simulink model "sm_car_"  (R2026b)
settings: Solver=ode23t  StopTime=100  MaxStep=0.4  AbsTol=1e-3  EnableMultiTasking=on
PreLoadFcn:
  | % Due to usability issue in Repeating Sequence block
  | warning('off','Simulink:Masking:Invalid');
  | 
  | % Eliminate unnecessary warnings in inactive variants
  | % Warnings generated only if you click through inactive variant
  | warning('off','MATLAB:nonExistentField');
  | warning('off','Simulink:Parameters:BlkParamUndefined');
PostLoadFcn:
  | set_param([bdroot '/Vehicle'],'popup_trailer','Off')
  | warning('off','sm:sli:setup:compile:LocalSolverNotSupported')
  | %sm_car_config_maneuver(bdroot,'WOT Braking');
  | sm_car_config_vehicle(bdroot,'false');
  | sm_car_config_logging(bdroot);
InitFcn:
  | sm_car_config_camera;
  | Vehicle = sm_car_vehcfg_checkConfig(Vehicle);
  | sm_car_check_tire_model(bdroot);
StartFcn:
  | tic;
StopFcn:
  | Elapsed_Sim_Time = toc;
  | % disp(['Elapsed Sim Time = ' num2str(Elapsed_Sim_Time)]);
undefined symbols (not defined in the file or in its folder): acc_theta, accel_ramp_rate, Axle1D, AxleIn, Camera, Control, Driver, Init, Maneuver, Pedal, Scene, ShaftL1, ShaftL2, ShaftR1, ShaftR2, Visual, X, xy_data_car_side, Y, Z
libraries: sm_lib x290, fl_lib x171, nesl_utility x144, simulink x60, simulink_extras x14, sdl_lib x14, SimscapeFluids_lib x7, Damper_Element x4, Tire_1x2x x4, ee_lib x3, Scene_Utilities x3, sharedTrackingLibrary x2
(part 10 of 22)

== system sm_car_/Driver/Closed Loop1/Override/None ==
  dist : Inport
  Obs : Inport  Port=2
  Bus Creator{,2..4} (4 alike) : BusCreator  Inputs=2
  Bus Creator1 : BusCreator  Inputs=4
  Constant{1..2,4,6} (4 alike) : Constant  Value=0
  Constant{3,5,7..8} (4 alike) : Constant
  Terminator : Terminator
  Terminator1 : Terminator
  Ovr : Outport  VectorParamsAs1DForOutWhenUnconnected=off
  wires:
  dist/1 -> Terminator/1
  Obs/1 -> Terminator1/1
  Bus Creator1/1 -> Ovr/1
  Constant1/1 -> Bus Creator/1  "offset"
  Constant8/1 -> Bus Creator/2  "gain"
  Constant6/1 -> Bus Creator4/1  "offset"
  Constant7/1 -> Bus Creator4/2  "gain"
  Constant5/1 -> Bus Creator3/2  "gain"
  Constant4/1 -> Bus Creator3/1  "offset"
  Constant3/1 -> Bus Creator2/2  "gain"
  Bus Creator2/1 -> Bus Creator1/3  "z"
  Constant2/1 -> Bus Creator2/1  "offset"
  Bus Creator3/1 -> Bus Creator1/2  "y"
  Bus Creator/1 -> Bus Creator1/4  "vx"
  Bus Creator4/1 -> Bus Creator1/1  "x"

== system sm_car_/Vehicle/Vehicle/Body to World/R to X-Y-Z Extrinsic ==
  note: The sensor implemented here computes roll / pitch / yaw values assuming they correpsond to X, Y, and Z rotations, applied in that order and using  *extrinsic* rotations.  That is, the rotations are applied about the fixed (non-rotated) axes of the base frame.   There are many other possible conventions, but the computations of angles has the same basic structure for any of them.  The only differences would be which elements of the rotation matrix are picked off for analysis, and which signals are negated.
      |
      | This implementation does not handle the gimbal-lock case robustly, which occurs when the Y (pitch) rotation is +/-90 degrees.  Handling this case requires a more complex computation,
      | but it can be done with a few more trig blocks and selectors.
  R : Inport
  Asin : Trigonometry  Operator=asin
  Atan1 : Trigonometry  Operator=atan2
  Atan2 : Trigonometry  Operator=atan2
  Demux : Demux  Outputs=2
  Demux1 : Demux  Outputs=2
  Multiply2 : Gain  Gain=-1
  "R(3, 1)" : Selector  NumberOfDimensions=2  InputPortWidth=3  IndexOptions=Index vector (dialog),Index vector (dialog)  Indices=3,1  OutputSizes=1,1  RuntimeRangeChecks=off
  "R(3, 2:3)" : Selector  NumberOfDimensions=2  InputPortWidth=3  IndexOptions=Index vector (dialog),Index vector (dialog)  Indices=3,[2 3]  OutputSizes=1,1  RuntimeRangeChecks=off
  "R([2 1], 1)" : Selector  NumberOfDimensions=2  InputPortWidth=3  IndexOptions=Index vector (dialog),Index vector (dialog)  Indices=[2 1],1  OutputSizes=1,1  RuntimeRangeChecks=off
  Reshape : Reshape
  Reshape1 : Reshape
  Reshape2 : Reshape  OutputDimensionality=Customize  OutputDimensions=1
  yaw : Outport  VectorParamsAs1DForOutWhenUnconnected=off
  pitch : Outport  Port=2  VectorParamsAs1DForOutWhenUnconnected=off
  roll : Outport  Port=3  VectorParamsAs1DForOutWhenUnconnected=off
  wires:
  Reshape2/1 -> roll/1
  Reshape1/1 -> pitch/1
  Reshape/1 -> yaw/1
  Atan1/1 -> Reshape/1
  "R(3, 2:3)"/1 -> Demux/1
  Multiply2/1 -> Asin/1
  "R([2 1], 1)"/1 -> Demux1/1
  Demux1/1 -> Atan1/1
  R/1 -> "R([2 1], 1)"/1, "R(3, 2:3)"/1, "R(3, 1)"/1
  Asin/1 -> Reshape1/1
  "R(3, 1)"/1 -> Multiply2/1
  Atan2/1 -> Reshape2/1
  Demux/2 -> Atan2/2
  Demux1/2 -> Atan1/2
  Demux/1 -> Atan2/1

== system sm_car_/Vehicle/Vehicle/Brakes/PedalAbstract DiscDisc ==
  In Bus Element5 : Inport  PortName=DrvBus  Element=rBrakePedal
  In Bus Element1 : Inport  Port=2  PortName=CtrlBus
  Actuator L1 : Subsystem  mask(Brake Actuator, Pedal Input){brk_max_p=brk_max_p_a1, brk_filt=brk_filt_a1}
      mask prompts: brk_max_p "Max Pad Pressure (Pa)"; brk_filt "Time Constant (s)"
      mask help: Models brake actuator dynamics. A transfer function models delay from brake pedal movement to pressure applied at brake rotor.
      mask TypeOptions brk_max_p: Filter/Numerator
  Actuator L2 : Subsystem  mask(Brake Actuator, Pedal Input){brk_max_p=brk_max_p_a2, brk_filt=brk_filt_a2}
      mask prompts: brk_max_p "Max Pad Pressure (Pa)"; brk_filt "Time Constant (s)"
      mask help: Models brake actuator dynamics. A transfer function models delay from brake pedal movement to pressure applied at brake rotor.
      mask TypeOptions brk_max_p: Filter/Numerator
  Actuator R1 : Subsystem  mask(Brake Actuator, Pedal Input){brk_max_p=brk_max_p_a1, brk_filt=brk_filt_a1}
      mask prompts: brk_max_p "Max Pad Pressure (Pa)"; brk_filt "Time Constant (s)"
      mask help: Models brake actuator dynamics. A transfer function models delay from brake pedal movement to pressure applied at brake rotor.
      mask TypeOptions brk_max_p: Filter/Numerator
  Actuator R2 : Subsystem  mask(Brake Actuator, Pedal Input){brk_max_p=brk_max_p_a2, brk_filt=brk_filt_a2}
      mask prompts: brk_max_p "Max Pad Pressure (Pa)"; brk_filt "Time Constant (s)"
      mask help: Models brake actuator dynamics. A transfer function models delay from brake pedal movement to pressure applied at brake rotor.
      mask TypeOptions brk_max_p: Filter/Numerator
  Disc Brake L1 : sdl_lib/Brakes & Detents/Rotational/Disc Brake  r_mean=brk_pad_rad_a1 m  bore=brk_cyl_bore_a1 m  n_pads=brk_n_pads_a1  thermal_port=simscape.enum.thermaleffects.omit  mu_static=brk_mu_static_a1  mu_coulomb=brk_mu_kin_a1  temperature_TLU=[280, 300, 320] K  mu_static_TLU=[.9, .8, .7]  mu_coulomb_TLU=[.8, .7, .6]  brkwy_vel=brk_trans_vel_a1 rad/s  visc_coef=brk_visc_coef_a1 N*m/(rad/s)  thermal_mass=50 kJ/K  temperature_specify=off  temperature_priority=High  temperature=300 K  temperature_nominal_specify=off  temperature_nominal_value=1  temperature_nominal_unit=K
  Disc Brake L2 : sdl_lib/Brakes & Detents/Rotational/Disc Brake  r_mean=brk_pad_rad_a2 m  bore=brk_cyl_bore_a2 m  n_pads=brk_n_pads_a2  thermal_port=simscape.enum.thermaleffects.omit  mu_static=brk_mu_static_a2  mu_coulomb=brk_mu_kin_a2  temperature_TLU=[280, 300, 320] K  mu_static_TLU=[.9, .8, .7]  mu_coulomb_TLU=[.8, .7, .6]  brkwy_vel=brk_trans_vel_a2 rad/s  visc_coef=brk_visc_coef_a2 N*m/(rad/s)  thermal_mass=50 kJ/K  temperature_specify=off  temperature_priority=High  temperature=300 K  temperature_nominal_specify=off  temperature_nominal_value=1  temperature_nominal_unit=K
  Disc Brake R1 : sdl_lib/Brakes & Detents/Rotational/Disc Brake  r_mean=brk_pad_rad_a1 m  bore=brk_cyl_bore_a1 m  n_pads=brk_n_pads_a1  thermal_port=simscape.enum.thermaleffects.omit  mu_static=brk_mu_static_a1  mu_coulomb=brk_mu_kin_a1  temperature_TLU=[280, 300, 320] K  mu_static_TLU=[.9, .8, .7]  mu_coulomb_TLU=[.8, .7, .6]  brkwy_vel=brk_trans_vel_a1 rad/s  visc_coef=brk_visc_coef_a1 N*m/(rad/s)  thermal_mass=50 kJ/K  temperature_specify=off  temperature_priority=High  temperature=300 K  temperature_nominal_specify=off  temperature_nominal_value=1  temperature_nominal_unit=K
  Disc Brake R2 : sdl_lib/Brakes & Detents/Rotational/Disc Brake  r_mean=brk_pad_rad_a2 m  bore=brk_cyl_bore_a2 m  n_pads=brk_n_pads_a2  thermal_port=simscape.enum.thermaleffects.omit  mu_static=brk_mu_static_a2  mu_coulomb=brk_mu_kin_a2  temperature_TLU=[280, 300, 320] K  mu_static_TLU=[.9, .8, .7]  mu_coulomb_TLU=[.8, .7, .6]  brkwy_vel=brk_trans_vel_a2 rad/s  visc_coef=brk_visc_coef_a2 N*m/(rad/s)  thermal_mass=50 kJ/K  temperature_specify=off  temperature_priority=High  temperature=300 K  temperature_nominal_specify=off  temperature_nominal_value=1  temperature_nominal_unit=K
  Sensing Torque L1 : Subsystem
  Sensing Torque L2 : Subsystem
  Sensing Torque R1 : Subsystem
  Sensing Torque R2 : Subsystem
  Simscape Bus L1 : SimscapeBus  HierarchyStrings=Axle1D
  Simscape Bus L2 : SimscapeBus  HierarchyStrings=Axle1D
  Simscape Bus R1 : SimscapeBus  HierarchyStrings=Axle1D
  Simscape Bus R2 : SimscapeBus  HierarchyStrings=Axle1D
  Terminator : Terminator
  L1 : PMIOPort  Side=Left
  R1 : PMIOPort  Port=2  Side=Right
  L2 : PMIOPort  Port=3  Side=Left
  R2 : PMIOPort  Port=4  Side=Right
  Out Bus Element2 : Outport  VectorParamsAs1DForOutWhenUnconnected=off  PortName=OutB  Element=MBrakeL1
  Out Bus Element : Outport  VectorParamsAs1DForOutWhenUnconnected=off  PortName=OutB  Element=MBrakeR1
  Out Bus Element3 : Outport  VectorParamsAs1DForOutWhenUnconnected=off  PortName=OutB  Element=MBrakeL2
  Out Bus Element4 : Outport  VectorParamsAs1DForOutWhenUnconnected=off  PortName=OutB  Element=MBrakeR2
  wires:
  In Bus Element5/1 -> Actuator L1/1(Pedal), Actuator R1/1(Pedal), Actuator R2/1(Pedal), Actuator L2/1(Pedal)
  In Bus Element1/1 -> Terminator/1
  Sensing Torque L1/1(T) -> Out Bus Element2/1
  Sensing Torque R1/1(T) -> Out Bus Element/1
  Sensing Torque L2/1(T) -> Out Bus Element3/1
  Sensing Torque R2/1(T) -> Out Bus Element4/1
  connections:
  Sensing Torque R2/LConn1 -- Disc Brake R2/LConn2
  Sensing Torque R1/LConn1 -- Disc Brake R1/LConn2
  Actuator R1/RConn1 -- Disc Brake R1/LConn1
  Actuator L2/RConn1 -- Disc Brake L2/LConn1
  Actuator L1/RConn1 -- Disc Brake L1/LConn1
  Actuator R2/RConn1 -- Disc Brake R2/LConn1
  R1/RConn1 -- Simscape Bus R1/RConn1
  R2/RConn1 -- Simscape Bus R2/RConn1
  Simscape Bus L2/RConn1 -- L2/RConn1
  Sensing Torque L2/LConn1 -- Disc Brake L2/LConn2
  Simscape Bus L1/RConn1 -- L1/RConn1
  Sensing Torque L1/LConn1 -- Disc Brake L1/LConn2
  Sensing Torque L1/RConn1 -- Simscape Bus L1/LConn1
  Sensing Torque R1/RConn1 -- Simscape Bus R1/LConn1
  Sensing Torque L2/RConn1 -- Simscape Bus L2/LConn1
  Sensing Torque R2/RConn1 -- Simscape Bus R2/LConn1

== system sm_car_/Vehicle/Vehicle/Chassis/Aero ==
  note: Lift force acts along the z axis of the frame where the External Force and Torque is attached. Direction is set by the Lift Coefficient.
  note: Drag force acts in the opposite direction of the x-velocity along the x axis of the frame where the External Force and Torque is attached
  fWind : Inport
  External Force Drag and Lift : sm_lib/Forces and Torques/External Force and Torque  EnableForceX=on  EnableForceY=off  EnableForceZ=on  EnableForce=off  ForceResolutionFrame=AttachedFrame  EnableTorqueX=off  EnableTorqueY=off  EnableTorqueZ=off  EnableTorque=off  TorqueResolutionFrame=AttachedFrame
  External Force Wind Gust : sm_lib/Forces and Torques/External Force and Torque  EnableForceX=off  EnableForceY=off  EnableForceZ=off  EnableForce=on  ForceResolutionFrame=World  EnableTorqueX=off  EnableTorqueY=off  EnableTorqueZ=off  EnableTorque=off  TorqueResolutionFrame=AttachedFrame
  Gain : Gain  Gain=0.5 * rho * CL * A
  Gain1 : Gain  Gain=-0.5 * rho * CD * A
  PS-Simulink Converter2 : nesl_utility/PS-Simulink Converter  PhysicalDomain=network_engine_domain  SubClassName=ps_output  LeftPortType=input  RightPortType=output  PseudoPeriodic=off  Frequencies=[]  VectorFormat=1-D array  Unit=1  AffineConversion=off
  Product : Product
  Product1 : Product
  Sign : Signum  ZeroCross=off
  Simulink-PS Converter : nesl_utility/Simulink-PS Converter  PhysicalDomain=network_engine_domain  SubClassName=ps_input  LeftPortType=input  RightPortType=output  PseudoPeriodic=off  Frequencies=[]  NoiseDistribution=none  NoiseParameters=[]  Unit=1  AffineConversion=off  FilteringAndDerivatives=provide  SimscapeFilterOrder=1  InputFilterTimeConstant=0.001  UdotUserProvided=0
  Simulink-PS Converter1 : nesl_utility/Simulink-PS Converter  PhysicalDomain=network_engine_domain  SubClassName=ps_input  LeftPortType=input  RightPortType=output  PseudoPeriodic=off  Frequencies=[]  NoiseDistribution=none  NoiseParameters=[]  Unit=1  AffineConversion=off  FilteringAndDerivatives=provide  SimscapeFilterOrder=1  InputFilterTimeConstant=0.001  UdotUserProvided=0
  Subsystem : Subsystem
  Transform Center of Pressure : sm_lib/Frames and Transforms/Rigid Transform  RotationMethod=None  FollAlignAxisA=+X  BaseAlignAxisA=+Y  FollAlignAxisB=+Y  BaseAlignAxisB=+Z  RotationStandardAxis=+Z  RotationAngle=0.0  RotationAngleUnits=deg  RotationArbitraryAxis=[0 0 1]  RotationSequenceAxes=FollowerAxes  RotationSequence=XYX  RotationSequenceAngles=[0 0 0]  RotationSequenceAnglesUnits=deg  RotationMatrix=[1 0 0; 0 1 0; 0 0 1]  Quaternion=[1 0 0 0]  TranslationMethod=Cartesian  TranslationCartesianOffset=sCentreOfPressure  TranslationCartesianOffsetUnits=m  TranslationStandardAxis=+Z  TranslationStandardOffset=0  TranslationStandardOffsetUnits=m  TranslationROffset=0  TranslationROffsetUnits=m  TranslationThetaOffset=0  TranslationThetaOffsetUnits=deg  TranslationZOffset=0  TranslationZOffsetUnits=m
  Transform Sensor : sm_lib/Frames and Transforms/Transform Sensor  ObservationFrame=World  ExpressedInFrame=Follower  RotationSequence=XYX  SenseAngle=off  SenseAxis=off  SenseQ=off  SenseR=off  SenseRotationSequence=off  SenseOmegaX=off  SenseOmegaY=off  SenseOmegaZ=off  SenseOmega=off  SenseQDot=off  SenseRDot=off  SenseRotationSequenceDot=off  SenseAlphaX=off  SenseAlphaY=off  SenseAlphaZ=off  SenseAlpha=off  SenseQDDot=off  SenseRDDot=off  SenseX=off  SenseY=off  SenseZ=off  SenseXYZ=off  SenseRad=off  SenseAzim=off  SenseDist=off  SenseInc=off  SenseXDot=on  SenseYDot=off  SenseZDot=off  SenseXYZDot=off  SenseRadDot=off  SenseAzimDot=off  SenseDistDot=off  SenseIncDot=off  SenseXDDot=off  SenseYDDot=off  SenseZDDot=off  SenseXYZDDot=off  SenseRadDDot=off  SenseAzimDDot=off  SenseDistDDot=off  SenseIncDDot=off
  Vis Center of Pressure : sm_lib/Body Elements/Spherical Solid  SphereRadius=rad_hp  SphereRadiusUnits=m  ExportEntireGeometry=off  InertiaType=CalculateFromGeometry  BasedOnType=Density  Density=1000  DensityUnits=kg/m^3  Mass=1  MassUnits=kg  CenterOfMass=[0 0 0]  CenterOfMassUnits=m  MomentsOfInertia=[1 1 1]  MomentsOfInertiaUnits=kg*m^2  ProductsOfInertia=[0 0 0]  ProductsOfInertiaUnits=kg*m^2  GraphicType=FromGeometry  MarkerShape=Sphere  MarkerSize=10  GraphicVisPropType=SimpleVisualProperties  GraphicDiffuseColor=clr_hp  GraphicOpacity=opc_hp  GraphicSpecularColor=[0.5 0.5 0.5 1.0]  GraphicAmbientColor=[0.15 0.15 0.15 1.0]  GraphicEmissiveColor=[0.0 0.0 0.0 1.0]  GraphicShininess=75  DoExposeReferenceFrame=on  SerializedFrames=<Frames/>
  World Frame : sm_lib/Frames and Transforms/World Frame
  A : PMIOPort  Side=Right
  Bus Element Out1 : Outport  VectorParamsAs1DForOutWhenUnconnected=off  PortName=meas  Element=Fx
  Bus Element Out : Outport  VectorParamsAs1DForOutWhenUnconnected=off  PortName=meas  Element=Fz
  wires:
  PS-Simulink Converter2/1 -> Product/1, Product/2, Sign/1
  Product1/1 -> Gain1/1
  Product/1 -> Gain/1, Product1/1
  Sign/1 -> Product1/2
  fWind/1 -> Subsystem/1(RdBus)
  Gain/1 -> Simulink-PS Converter/1, Bus Element Out/1
  Gain1/1 -> Simulink-PS Converter1/1, Bus Element Out1/1
  connections:
  Simulink-PS Converter/RConn1 -- External Force Drag and Lift/LConn2
  Simulink-PS Converter1/RConn1 -- External Force Drag and Lift/LConn1
  Subsystem/RConn1 -- External Force Wind Gust/LConn1
  Transform Center of Pressure/RConn1 -- Vis Center of Pressure/RConn1 -- External Force Wind Gust/RConn1 -- Transform Sensor/RConn1 -- External Force Drag and Lift/RConn1
  Transform Center of Pressure/LConn1 -- A/RConn1
  PS-Simulink Converter2/LConn1 -- Transform Sensor/RConn2
  Transform Sensor/LConn1 -- World Frame/RConn1

== system sm_car_/Vehicle/Vehicle/Chassis/Body ==
  Body Geometry : Subsystem  Variant=on  VariantControlMode=label  VariantControl=Variant1  LabelModeActiveChoice=CAD_FSAE_Achilles  mask(Variants for Vehicle Body Geometry){BodyGeometry=BodyGeometry, VariantLabel=BodyGeometry.class.Value}
      mask prompts: VariantLabel "Variant Label"
      mask help: Select option and provide parameters for vehicle body geometry. Option is chosen by string provided in Variant Label. The parameters for the selected option is contained in Body Geometry data structure.
      mask init:
      | curblk = gcb;
      | 
      | % Set variant for this block 
      | set_param(curblk,'LabelModeActiveChoice',VariantLabel);
      settings: AttributesFormatString=%<LabelModeActiveChoice>
  Body Load : Subsystem  Variant=on  VariantControlMode=label  VariantControl=Variant1  LabelModeActiveChoice=None  mask(Variants for Vehicle Body Load){BodyLoad=BodyLoad, VariantLabel=BodyLoad.class.Value}
      mask prompts: VariantLabel "Variant Label"
      mask help: Select option and provide parameters for vehicle body load. Option is chosen by string provided in Variant Label. The parameters for the selected option is contained in Body Load data structure.
      mask init:
      | curblk = gcb;
      | 
      | % Set variant for this block 
      | set_param(curblk,'LabelModeActiveChoice',VariantLabel);
      settings: AttributesFormatString=%<LabelModeActiveChoice>
  Body Mass and Inertia : sm_lib/Body Elements/Spherical Solid  SphereRadius=size_chassis_hp_cg  SphereRadiusUnits=m  ExportEntireGeometry=off  InertiaType=Custom  BasedOnType=Density  Density=312*0.6  DensityUnits=kg/m^3  Mass=chassis_mass  MassUnits=kg  CenterOfMass=[0 0 0]  CenterOfMassUnits=m  MomentsOfInertia=chassis_inertia  MomentsOfInertiaUnits=kg*m^2  ProductsOfInertia=[0 0 0]  ProductsOfInertiaUnits=kg*m^2  GraphicType=FromGeometry  MarkerShape=Sphere  MarkerSize=10  GraphicVisPropType=SimpleVisualProperties  GraphicDiffuseColor=clr_chassis_hp_cg  GraphicOpacity=opc_chassis_hp_cg  GraphicSpecularColor=[0.5 0.5 0.5 1.0]  GraphicAmbientColor=[0.15 0.15 0.15 1.0]  GraphicEmissiveColor=[0.0 0.0 0.0 1.0]  GraphicShininess=75  DoExposeReferenceFrame=on  SerializedFrames=<Frames/>
  Body Sensor : Subsystem  mask{offset_body_sensor=[0 0 0]}
      mask prompts: offset_body_sensor "Sensor Frame Offset [x y z] (m)"
  Reference Frame Front Hitch : sm_lib/Frames and Transforms/Reference Frame
  Reference Frame Rear Hitch : sm_lib/Frames and Transforms/Reference Frame
  Transform Body CG : sm_lib/Frames and Transforms/Rigid Transform  RotationMethod=None  FollAlignAxisA=+X  BaseAlignAxisA=+Y  FollAlignAxisB=+Y  BaseAlignAxisB=+Z  RotationStandardAxis=+Z  RotationAngle=0.0  RotationAngleUnits=deg  RotationArbitraryAxis=[0 0 1]  RotationSequenceAxes=FollowerAxes  RotationSequence=XYX  RotationSequenceAngles=[0 0 0]  RotationSequenceAnglesUnits=deg  RotationMatrix=[1 0 0; 0 1 0; 0 0 1]  Quaternion=[1 0 0 0]  TranslationMethod=Cartesian  TranslationCartesianOffset=hp_chassis_cg  TranslationCartesianOffsetUnits=m  TranslationStandardAxis=+Z  TranslationStandardOffset=0  TranslationStandardOffsetUnits=m  TranslationROffset=0  TranslationROffsetUnits=m  TranslationThetaOffset=0  TranslationThetaOffsetUnits=deg  TranslationZOffset=0  TranslationZOffsetUnits=m
  Transform Front Hitch : sm_lib/Frames and Transforms/Rigid Transform  RotationMethod=None  FollAlignAxisA=+X  BaseAlignAxisA=+Y  FollAlignAxisB=+Y  BaseAlignAxisB=+Z  RotationStandardAxis=+Z  RotationAngle=0.0  RotationAngleUnits=deg  RotationArbitraryAxis=[0 0 1]  RotationSequenceAxes=FollowerAxes  RotationSequence=XYX  RotationSequenceAngles=[0 0 0]  RotationSequenceAnglesUnits=deg  RotationMatrix=[1 0 0; 0 1 0; 0 0 1]  Quaternion=[1 0 0 0]  TranslationMethod=Cartesian  TranslationCartesianOffset=hp_mount_hitchf  TranslationCartesianOffsetUnits=m  TranslationStandardAxis=-X  TranslationStandardOffset=0  TranslationStandardOffsetUnits=m  TranslationROffset=0  TranslationROffsetUnits=m  TranslationThetaOffset=0  TranslationThetaOffsetUnits=deg  TranslationZOffset=0  TranslationZOffsetUnits=m
  Transform Mount A1 : sm_lib/Frames and Transforms/Rigid Transform  RotationMethod=None  FollAlignAxisA=+X  BaseAlignAxisA=+Y  FollAlignAxisB=+Y  BaseAlignAxisB=+Z  RotationStandardAxis=+Z  RotationAngle=0.0  RotationAngleUnits=deg  RotationArbitraryAxis=[0 0 1]  RotationSequenceAxes=FollowerAxes  RotationSequence=XYX  RotationSequenceAngles=[0 0 0]  RotationSequenceAnglesUnits=deg  RotationMatrix=[1 0 0; 0 1 0; 0 0 1]  Quaternion=[1 0 0 0]  TranslationMethod=Cartesian  TranslationCartesianOffset=hp_mount_a1  TranslationCartesianOffsetUnits=m  TranslationStandardAxis=+X  TranslationStandardOffset=0  TranslationStandardOffsetUnits=m  TranslationROffset=0  TranslationROffsetUnits=m  TranslationThetaOffset=0  TranslationThetaOffsetUnits=deg  TranslationZOffset=0  TranslationZOffsetUnits=m
  Transform Mount A2 : sm_lib/Frames and Transforms/Rigid Transform  RotationMethod=None  FollAlignAxisA=+X  BaseAlignAxisA=+Y  FollAlignAxisB=+Y  BaseAlignAxisB=+Z  RotationStandardAxis=+Z  RotationAngle=0.0  RotationAngleUnits=deg  RotationArbitraryAxis=[0 0 1]  RotationSequenceAxes=FollowerAxes  RotationSequence=XYX  RotationSequenceAngles=[0 0 0]  RotationSequenceAnglesUnits=deg  RotationMatrix=[1 0 0; 0 1 0; 0 0 1]  Quaternion=[1 0 0 0]  TranslationMethod=Cartesian  TranslationCartesianOffset=hp_mount_a2  TranslationCartesianOffsetUnits=m  TranslationStandardAxis=-X  TranslationStandardOffset=0  TranslationStandardOffsetUnits=m  TranslationROffset=0  TranslationROffsetUnits=m  TranslationThetaOffset=0  TranslationThetaOffsetUnits=deg  TranslationZOffset=0  TranslationZOffsetUnits=m
  Transform Power Mount : sm_lib/Frames and Transforms/Rigid Transform  RotationMethod=None  FollAlignAxisA=+X  BaseAlignAxisA=+Y  FollAlignAxisB=+Y  BaseAlignAxisB=+Z  RotationStandardAxis=+Z  RotationAngle=0.0  RotationAngleUnits=deg  RotationArbitraryAxis=[0 0 1]  RotationSequenceAxes=FollowerAxes  RotationSequence=XYX  RotationSequenceAngles=[0 0 0]  RotationSequenceAnglesUnits=deg  RotationMatrix=[1 0 0; 0 1 0; 0 0 1]  Quaternion=[1 0 0 0]  TranslationMethod=Cartesian  TranslationCartesianOffset=hp_mount_power  TranslationCartesianOffsetUnits=m  TranslationStandardAxis=+Z  TranslationStandardOffset=0  TranslationStandardOffsetUnits=m  TranslationROffset=0  TranslationROffsetUnits=m  TranslationThetaOffset=0  TranslationThetaOffsetUnits=deg  TranslationZOffset=0  TranslationZOffsetUnits=m
  Transform Rear Hitch : sm_lib/Frames and Transforms/Rigid Transform  RotationMethod=None  FollAlignAxisA=+X  BaseAlignAxisA=+Y  FollAlignAxisB=+Y  BaseAlignAxisB=+Z  RotationStandardAxis=+Z  RotationAngle=0.0  RotationAngleUnits=deg  RotationArbitraryAxis=[0 0 1]  RotationSequenceAxes=FollowerAxes  RotationSequence=XYX  RotationSequenceAngles=[0 0 0]  RotationSequenceAnglesUnits=deg  RotationMatrix=[1 0 0; 0 1 0; 0 0 1]  Quaternion=[1 0 0 0]  TranslationMethod=Cartesian  TranslationCartesianOffset=hp_mount_hitchr  TranslationCartesianOffsetUnits=m  TranslationStandardAxis=-X  TranslationStandardOffset=0  TranslationStandardOffsetUnits=m  TranslationROffset=0  TranslationROffsetUnits=m  TranslationThetaOffset=0  TranslationThetaOffsetUnits=deg  TranslationZOffset=0  TranslationZOffsetUnits=m
  Vis HP Mount A1 : sm_lib/Body Elements/Spherical Solid  SphereRadius=size_chassis_hp_cg  SphereRadiusUnits=m  ExportEntireGeometry=off  InertiaType=PointMass  BasedOnType=Density  Density=312*0.6  DensityUnits=kg/m^3  Mass=0  MassUnits=kg  CenterOfMass=[0 0 0]  CenterOfMassUnits=m  MomentsOfInertia=[1 1 1]  MomentsOfInertiaUnits=kg*m^2  ProductsOfInertia=[0 0 0]  ProductsOfInertiaUnits=kg*m^2  GraphicType=FromGeometry  MarkerShape=Sphere  MarkerSize=10  GraphicVisPropType=SimpleVisualProperties  GraphicDiffuseColor=clr_chassis_hp_cg  GraphicOpacity=opc_chassis_hp_cg  GraphicSpecularColor=[0.5 0.5 0.5 1.0]  GraphicAmbientColor=[0.15 0.15 0.15 1.0]  GraphicEmissiveColor=[0.0 0.0 0.0 1.0]  GraphicShininess=75  DoExposeReferenceFrame=on  SerializedFrames=<Frames/>
  Vis HP Mount A2 : sm_lib/Body Elements/Spherical Solid  SphereRadius=size_chassis_hp_cg  SphereRadiusUnits=m  ExportEntireGeometry=off  InertiaType=PointMass  BasedOnType=Density  Density=312*0.6  DensityUnits=kg/m^3  Mass=0  MassUnits=kg  CenterOfMass=[0 0 0]  CenterOfMassUnits=m  MomentsOfInertia=[1 1 1]  MomentsOfInertiaUnits=kg*m^2  ProductsOfInertia=[0 0 0]  ProductsOfInertiaUnits=kg*m^2  GraphicType=FromGeometry  MarkerShape=Sphere  MarkerSize=10  GraphicVisPropType=SimpleVisualProperties  GraphicDiffuseColor=clr_chassis_hp_cg  GraphicOpacity=opc_chassis_hp_cg  GraphicSpecularColor=[0.5 0.5 0.5 1.0]  GraphicAmbientColor=[0.15 0.15 0.15 1.0]  GraphicEmissiveColor=[0.0 0.0 0.0 1.0]  GraphicShininess=75  DoExposeReferenceFrame=on  SerializedFrames=<Frames/>
  HF : PMIOPort  Side=Left
  A1 : PMIOPort  Port=2  Side=Right
  Pwr : PMIOPort  Port=3  Side=Left
  W : PMIOPort  Port=4  Side=Left
  A2 : PMIOPort  Port=5  Side=Right
  HR : PMIOPort  Port=6  Side=Left
  Out Bus Element1 : Outport  VectorParamsAs1DForOutWhenUnconnected=off  PortName=m  Element=CG
  wires:
  Body Sensor/1(Body) -> Out Bus Element1/1
  connections:
  Reference Frame Front Hitch/RConn1 -- Transform Front Hitch/RConn1 -- HF/RConn1
  Reference Frame Rear Hitch/RConn1 -- Transform Rear Hitch/RConn1 -- HR/RConn1
  Pwr/RConn1 -- Transform Power Mount/RConn1
  Transform Mount A2/RConn1 -- A2/RConn1 -- Vis HP Mount A2/RConn1
  Transform Mount A1/RConn1 -- Vis HP Mount A1/RConn1 -- A1/RConn1 -- Body Load/LConn1 -- Body Geometry/RConn1
  Transform Body CG/RConn1 -- Body Sensor/LConn1 -- Body Mass and Inertia/RConn1
  W/RConn1 -- Transform Rear Hitch/LConn1 -- Transform Front Hitch/LConn1 -- Transform Mount A1/LConn1 -- Transform Mount A2/LConn1 -- Transform Power Mount/LConn1 -- Transform Body CG/LConn1

== system sm_car_/Vehicle/Vehicle/Chassis/Damper ==
  "Ctrl " : Inport
  Decoupled : Subsystem  VariantControl=Decoupled  mask(Roll and Heave Dampers){}
      mask help: Models dampers in a suspension design that decouples damping for body roll and heave .
  Independent : Subsystem  VariantControl=Independent  mask(Independent Dampers){}
      mask help: Models independent left and right dampers on two axles
  " L1" : PMIOPort  Side=Left
  " R1" : PMIOPort  Port=2  Side=Right
  " L2" : PMIOPort  Port=3  Side=Left
  " R2" : PMIOPort  Port=4  Side=Right
  " meas" : Outport  VectorParamsAs1DForOutWhenUnconnected=off

== system sm_car_/Vehicle/Vehicle/Chassis/Spring ==
  "Ctrl " : Inport
  Decoupled : Subsystem  VariantControl=Decoupled  mask(Roll and Heave Springs){}
      mask help: Models springs in a suspension design that decouples stiffness for body roll and heave .
  Independent : Subsystem  VariantControl=Independent  mask(Independent Springs){}
      mask help: Models independent left and right springs on two axles
  " L1" : PMIOPort  Side=Left
  R1 : PMIOPort  Port=2  Side=Right
  " L2" : PMIOPort  Port=3  Side=Left
  R2 : PMIOPort  Port=4  Side=Right
  " meas" : Outport  VectorParamsAs1DForOutWhenUnconnected=off

== system sm_car_/Vehicle/Vehicle/Powertrain/Driveline ==
  CtrlBus : Inport
  L2 R2 : Subsystem  Tag=PublishSubsystem  VariantControl=L2_R2  mask(Driveline, Two-Axle, Four Input Shaft){}
      mask help: Models two-axle driveline with four separate shafts. The shafts are connected independently to the wheels.
      mask Display: image('sm_car_vehicle_driveline_axle2_l1_r1_l2_r2_IMAGE.png');
  A1 : PMIOPort  Side=Left
  A2 : PMIOPort  Port=2  Side=Right
  L1 : PMIOPort  Port=3  Side=Left
  R1 : PMIOPort  Port=4  Side=Right
  L2 : PMIOPort  Port=5  Side=Left
  R2 : PMIOPort  Port=6  Side=Right
  Shafts : PMIOPort  Port=7  Side=Left
  " o" : PMIOPort  Port=8  Side=Right
  OutD : Outport  VectorParamsAs1DForOutWhenUnconnected=off

== system sm_car_/Vehicle/Vehicle/Powertrain/Power ==
  CtrlBus : Inport
  VehBus : Inport  Port=2
  Electric L2 R2 : Subsystem  VariantControl=Electric_L2_R2  mask(Electric Propulsion with Four Motors){Power=Powertrain.Power}
      mask prompts: Power "Power 4 Motor (structure)"
      mask help: Four electric motors with optional cooling system. Physical connections for the four motor shafts are in bus Shafts.
      mask Display: image('sm_car_vehicle_power_e4motor_IMAGE.png');
  Shafts : PMIOPort  Side=Left
  Ref : PMIOPort  Port=2  Side=Right
  OutP : Outport  VectorParamsAs1DForOutWhenUnconnected=off

== system sm_car_/World/Scene/CRG Hockenheim/Finish Line ==
  L1 : Subsystem  mask{square_lwh=[0.01 1 1]}
      mask prompts: square_lwh "Size [l w h] (m)"
  L2 : Subsystem  mask{square_lwh=[0.01 1 1]}
      mask prompts: square_lwh "Size [l w h] (m)"
  L3 : Subsystem  mask{square_lwh=[0.01 1 1]}
      mask prompts: square_lwh "Size [l w h] (m)"
  L4 : Subsystem  mask{square_lwh=[0.01 1 1]}
      mask prompts: square_lwh "Size [l w h] (m)"
  L5 : Subsystem  mask{square_lwh=[0.01 1 1]}
      mask prompts: square_lwh "Size [l w h] (m)"
  Post L : sm_lib/Body Elements/Cylindrical Solid  CylinderRadius=post_r  CylinderRadiusUnits=m  CylinderLength=post_h  CylinderLengthUnits=m  ExportEntireGeometry=off  InertiaType=CalculateFromGeometry  BasedOnType=Density  Density=1000  DensityUnits=kg/m^3  Mass=1  MassUnits=kg  CenterOfMass=[0 0 0]  CenterOfMassUnits=m  MomentsOfInertia=[1 1 1]  MomentsOfInertiaUnits=kg*m^2  ProductsOfInertia=[0 0 0]  ProductsOfInertiaUnits=kg*m^2  GraphicType=FromGeometry  MarkerShape=Sphere  MarkerSize=10  GraphicVisPropType=SimpleVisualProperties  GraphicDiffuseColor=post_clr  GraphicOpacity=post_opc  GraphicSpecularColor=[0.5 0.5 0.5 1.0]  GraphicAmbientColor=[0.15 0.15 0.15 1.0]  GraphicEmissiveColor=[0.0 0.0 0.0 1.0]  GraphicShininess=75  DoExposeReferenceFrame=off  SerializedFrames=<Frames><Frame><Id>Frame1</Id><Value><Name>B</Name><Origin><Source>GeometricFeature</Source><FeatureName>bottom surface</FeatureName></Origin><PrimaryAxis><DefinedDirection>+Z</DefinedDirection><Source>ReferenceFrame</Source><SourceDirection>+Z</SourceDirection><FeatureName></FeatureName></PrimaryAxis><SecondaryAxis><DefinedDirection>+X</DefinedDirection><Source>ReferenceFrame</Source><SourceDirection>+X</SourceDirection><FeatureName></FeatureName></SecondaryAxis></Value></Frame><Frame><Id>Frame2</Id><Value><Name>T</Name><Origin><Source>GeometricFeature</Source><FeatureName>top surface</FeatureName></Origin><PrimaryAxis><DefinedDirection>+Z</DefinedDirection><Source>ReferenceFrame</Source><SourceDirection>+Z</SourceDirection><FeatureName></FeatureName></PrimaryAxis><SecondaryAxis><DefinedDirection>+X</DefinedDirection><Source>ReferenceFrame</Source><SourceDirection>+X</SourceDirection><FeatureName></FeatureName></SecondaryAxis></Value></Frame></Frames>
  Post R : sm_lib/Body Elements/Cylindrical Solid  CylinderRadius=post_r  CylinderRadiusUnits=m  CylinderLength=post_h  CylinderLengthUnits=m  ExportEntireGeometry=off  InertiaType=CalculateFromGeometry  BasedOnType=Density  Density=1000  DensityUnits=kg/m^3  Mass=1  MassUnits=kg  CenterOfMass=[0 0 0]  CenterOfMassUnits=m  MomentsOfInertia=[1 1 1]  MomentsOfInertiaUnits=kg*m^2  ProductsOfInertia=[0 0 0]  ProductsOfInertiaUnits=kg*m^2  GraphicType=FromGeometry  MarkerShape=Sphere  MarkerSize=10  GraphicVisPropType=SimpleVisualProperties  GraphicDiffuseColor=post_clr  GraphicOpacity=post_opc  GraphicSpecularColor=[0.5 0.5 0.5 1.0]  GraphicAmbientColor=[0.15 0.15 0.15 1.0]  GraphicEmissiveColor=[0.0 0.0 0.0 1.0]  GraphicShininess=75  DoExposeReferenceFrame=off  SerializedFrames=<Frames><Frame><Id>Frame1</Id><Value><Name>B</Name><Origin><Source>GeometricFeature</Source><FeatureName>bottom surface</FeatureName></Origin><PrimaryAxis><DefinedDirection>+Z</DefinedDirection><Source>ReferenceFrame</Source><SourceDirection>+Z</SourceDirection><FeatureName></FeatureName></PrimaryAxis><SecondaryAxis><DefinedDirection>+X</DefinedDirection><Source>ReferenceFrame</Source><SourceDirection>+X</SourceDirection><FeatureName></FeatureName></SecondaryAxis></Value></Frame><Frame><Id>Frame2</Id><Value><Name>T</Name><Origin><Source>GeometricFeature</Source><FeatureName>top surface</FeatureName></Origin><PrimaryAxis><DefinedDirection>+Z</DefinedDirection><Source>ReferenceFrame</Source><SourceDirection>+Z</SourceDirection><FeatureName></FeatureName></PrimaryAxis><SecondaryAxis><DefinedDirection>+X</DefinedDirection><Source>ReferenceFrame</Source><SourceDirection>+X</SourceDirection><FeatureName></FeatureName></SecondaryAxis></Value></Frame></Frames>
  R1 : Subsystem  mask{square_lwh=[0.01 1 1]}
      mask prompts: square_lwh "Size [l w h] (m)"
  R2 : Subsystem  mask{square_lwh=[0.01 1 1]}
      mask prompts: square_lwh "Size [l w h] (m)"
  R3 : Subsystem  mask{square_lwh=[0.01 1 1]}
      mask prompts: square_lwh "Size [l w h] (m)"
  R4 : Subsystem  mask{square_lwh=[0.01 1 1]}
      mask prompts: square_lwh "Size [l w h] (m)"
  R5 : Subsystem  mask{square_lwh=[0.01 1 1]}
      mask prompts: square_lwh "Size [l w h] (m)"
  Transform Orient Line : sm_lib/Frames and Transforms/Rigid Transform  RotationMethod=RotationSequence  FollAlignAxisA=+X  BaseAlignAxisA=+Y  FollAlignAxisB=+Y  BaseAlignAxisB=+Z  RotationStandardAxis=+Z  RotationAngle=0  RotationAngleUnits=deg  RotationArbitraryAxis=[0 0 1]  RotationSequenceAxes=FollowerAxes  RotationSequence=ZYX  RotationSequenceAngles=[offset_yaw offset_pitch offset_roll]  RotationSequenceAnglesUnits=rad  RotationMatrix=[1 0 0; 0 1 0; 0 0 1]  Quaternion=[1 0 0 0]  TranslationMethod=Cartesian  TranslationCartesianOffset=offset_xyz  TranslationCartesianOffsetUnits=m  TranslationStandardAxis=+Z  TranslationStandardOffset=0  TranslationStandardOffsetUnits=m  TranslationROffset=0  TranslationROffsetUnits=m  TranslationThetaOffset=0  TranslationThetaOffsetUnits=deg  TranslationZOffset=0  TranslationZOffsetUnits=m
  Transform Post L : sm_lib/Frames and Transforms/Rigid Transform  RotationMethod=StandardAxis  FollAlignAxisA=+X  BaseAlignAxisA=+Y  FollAlignAxisB=+Y  BaseAlignAxisB=+Z  RotationStandardAxis=+Y  RotationAngle=0.0  RotationAngleUnits=deg  RotationArbitraryAxis=[0 0 1]  RotationSequenceAxes=FollowerAxes  RotationSequence=XYX  RotationSequenceAngles=[0 0 0]  RotationSequenceAnglesUnits=deg  RotationMatrix=[1 0 0; 0 1 0; 0 0 1]  Quaternion=[1 0 0 0]  TranslationMethod=StandardAxis  TranslationCartesianOffset=[0 0 0]  TranslationCartesianOffsetUnits=m  TranslationStandardAxis=+Y  TranslationStandardOffset=line_w/2  TranslationStandardOffsetUnits=m  TranslationROffset=0  TranslationROffsetUnits=m  TranslationThetaOffset=0  TranslationThetaOffsetUnits=deg  TranslationZOffset=0  TranslationZOffsetUnits=m
  Transform Post R : sm_lib/Frames and Transforms/Rigid Transform  RotationMethod=StandardAxis  FollAlignAxisA=+X  BaseAlignAxisA=+Y  FollAlignAxisB=+Y  BaseAlignAxisB=+Z  RotationStandardAxis=+Y  RotationAngle=0.0  RotationAngleUnits=deg  RotationArbitraryAxis=[0 0 1]  RotationSequenceAxes=FollowerAxes  RotationSequence=XYX  RotationSequenceAngles=[0 0 0]  RotationSequenceAnglesUnits=deg  RotationMatrix=[1 0 0; 0 1 0; 0 0 1]  Quaternion=[1 0 0 0]  TranslationMethod=StandardAxis  TranslationCartesianOffset=[0 0 0]  TranslationCartesianOffsetUnits=m  TranslationStandardAxis=+Y  TranslationStandardOffset=line_w/2  TranslationStandardOffsetUnits=m  TranslationROffset=0  TranslationROffsetUnits=m  TranslationThetaOffset=0  TranslationThetaOffsetUnits=deg  TranslationZOffset=0  TranslationZOffsetUnits=m
  W : PMIOPort  Side=Left
  connections:
  Post R/RConn1 -- R1/RConn1
  R2/RConn1 -- R1/LConn1
  L2/RConn1 -- L3/LConn1
  R4/RConn1 -- R3/LConn1
  Transform Post R/LConn1 -- Post R/LConn1
  L3/RConn1 -- L4/LConn1
  Post L/LConn1 -- Transform Post L/RConn1
  W/RConn1 -- Transform Orient Line/LConn1
  R2/LConn1 -- R3/RConn1
  L5/LConn1 -- L4/RConn1
  R5/RConn1 -- R4/LConn1
  L1/RConn1 -- L2/LConn1
  L1/LConn1 -- Post L/RConn1
  Transform Post L/LConn1 -- Transform Orient Line/RConn1 -- Transform Post R/RConn1

== system sm_car_/World/Scene/CRG Hockenheim/STL Geometry Centerline ==
  Geometry : sm_lib/Body Elements/File Solid  ExtGeomFileName=CRG_Hockenheim_centerline.stl  UnitType=Custom  ExtGeomFileUnits=m  StepReaderType=HEX  ExportConvexHullGeometry=off  InertiaType=Custom  BasedOnType=DensityFromFile  Density=1000  DensityUnits=kg/m^3  Mass=1  MassUnits=kg  CenterOfMass=[0 0 0]  CenterOfMassUnits=m  MomentsOfInertia=[1 1 1]  MomentsOfInertiaUnits=kg*m^2  ProductsOfInertia=[0 0 0]  ProductsOfInertiaUnits=kg*m^2  GraphicType=FromGeometry  MarkerShape=Sphere  MarkerSize=10  GraphicVisPropType=SimpleVisualProperties  GraphicDiffuseColor=stl_clr  GraphicOpacity=stl_opc  GraphicSpecularColor=[0.5 0.5 0.5 1.0]  GraphicAmbientColor=[0.15 0.15 0.15 1.0]  GraphicEmissiveColor=[0.0 0.0 0.0 1.0]  GraphicShininess=75  DoExposeReferenceFrame=on  SerializedFrames=<Frames/>
  Transform Geometry : sm_lib/Frames and Transforms/Rigid Transform  RotationMethod=RotationSequence  FollAlignAxisA=+X  BaseAlignAxisA=+Y  FollAlignAxisB=+Y  BaseAlignAxisB=+Z  RotationStandardAxis=+Z  RotationAngle=0  RotationAngleUnits=rad  RotationArbitraryAxis=[0 0 1]  RotationSequenceAxes=FollowerAxes  RotationSequence=ZYX  RotationSequenceAngles=[stl_yaw stl_pitch stl_roll]  RotationSequenceAnglesUnits=rad  RotationMatrix=[1 0 0; 0 1 0; 0 0 1]  Quaternion=[1 0 0 0]  TranslationMethod=Cartesian  TranslationCartesianOffset=[stl_x stl_y stl_z]  TranslationCartesianOffsetUnits=m  TranslationStandardAxis=+Z  TranslationStandardOffset=0  TranslationStandardOffsetUnits=m  TranslationROffset=0  TranslationROffsetUnits=m  TranslationThetaOffset=0  TranslationThetaOffsetUnits=deg  TranslationZOffset=0  TranslationZOffsetUnits=m
  W : PMIOPort  Side=Right
  connections:
  Geometry/RConn1 -- Transform Geometry/RConn1
  Transform Geometry/LConn1 -- W/RConn1

== system sm_car_/World/Scene/CRG Hockenheim/STL Geometry Road ==
  Geometry : sm_lib/Body Elements/File Solid  ExtGeomFileName=CRG_Hockenheim.stl  UnitType=Custom  ExtGeomFileUnits=m  StepReaderType=HEX  ExportConvexHullGeometry=off  InertiaType=Custom  BasedOnType=DensityFromFile  Density=1000  DensityUnits=kg/m^3  Mass=1  MassUnits=kg  CenterOfMass=[0 0 0]  CenterOfMassUnits=m  MomentsOfInertia=[1 1 1]  MomentsOfInertiaUnits=kg*m^2  ProductsOfInertia=[0 0 0]  ProductsOfInertiaUnits=kg*m^2  GraphicType=FromGeometry  MarkerShape=Sphere  MarkerSize=10  GraphicVisPropType=SimpleVisualProperties  GraphicDiffuseColor=stl_clr  GraphicOpacity=stl_opc  GraphicSpecularColor=[0.5 0.5 0.5 1.0]  GraphicAmbientColor=[0.15 0.15 0.15 1.0]  GraphicEmissiveColor=[0.0 0.0 0.0 1.0]  GraphicShininess=75  DoExposeReferenceFrame=on  SerializedFrames=<Frames/>
  Transform Geometry : sm_lib/Frames and Transforms/Rigid Transform  RotationMethod=RotationSequence  FollAlignAxisA=+X  BaseAlignAxisA=+Y  FollAlignAxisB=+Y  BaseAlignAxisB=+Z  RotationStandardAxis=+Z  RotationAngle=0  RotationAngleUnits=rad  RotationArbitraryAxis=[0 0 1]  RotationSequenceAxes=FollowerAxes  RotationSequence=ZYX  RotationSequenceAngles=[stl_yaw stl_pitch stl_roll]  RotationSequenceAnglesUnits=rad  RotationMatrix=[1 0 0; 0 1 0; 0 0 1]  Quaternion=[1 0 0 0]  TranslationMethod=Cartesian  TranslationCartesianOffset=[stl_x stl_y stl_z]  TranslationCartesianOffsetUnits=m  TranslationStandardAxis=+Z  TranslationStandardOffset=0  TranslationStandardOffsetUnits=m  TranslationROffset=0  TranslationROffsetUnits=m  TranslationThetaOffset=0  TranslationThetaOffsetUnits=deg  TranslationZOffset=0  TranslationZOffsetUnits=m
  W : PMIOPort  Side=Right
  connections:
  Geometry/RConn1 -- Transform Geometry/RConn1
  Transform Geometry/LConn1 -- W/RConn1

== system sm_car_/World/Scene/CRG Hockenheim F/Finish Line ==
  L1 : Subsystem  mask{square_lwh=[0.01 1 1]}
      mask prompts: square_lwh "Size [l w h] (m)"
  L2 : Subsystem  mask{square_lwh=[0.01 1 1]}
      mask prompts: square_lwh "Size [l w h] (m)"
  L3 : Subsystem  mask{square_lwh=[0.01 1 1]}
      mask prompts: square_lwh "Size [l w h] (m)"
  L4 : Subsystem  mask{square_lwh=[0.01 1 1]}
      mask prompts: square_lwh "Size [l w h] (m)"
  L5 : Subsystem  mask{square_lwh=[0.01 1 1]}
      mask prompts: square_lwh "Size [l w h] (m)"
  Post L : sm_lib/Body Elements/Cylindrical Solid  CylinderRadius=post_r  CylinderRadiusUnits=m  CylinderLength=post_h  CylinderLengthUnits=m  ExportEntireGeometry=off  InertiaType=CalculateFromGeometry  BasedOnType=Density  Density=1000  DensityUnits=kg/m^3  Mass=1  MassUnits=kg  CenterOfMass=[0 0 0]  CenterOfMassUnits=m  MomentsOfInertia=[1 1 1]  MomentsOfInertiaUnits=kg*m^2  ProductsOfInertia=[0 0 0]  ProductsOfInertiaUnits=kg*m^2  GraphicType=FromGeometry  MarkerShape=Sphere  MarkerSize=10  GraphicVisPropType=SimpleVisualProperties  GraphicDiffuseColor=post_clr  GraphicOpacity=post_opc  GraphicSpecularColor=[0.5 0.5 0.5 1.0]  GraphicAmbientColor=[0.15 0.15 0.15 1.0]  GraphicEmissiveColor=[0.0 0.0 0.0 1.0]  GraphicShininess=75  DoExposeReferenceFrame=off  SerializedFrames=<Frames><Frame><Id>Frame1</Id><Value><Name>B</Name><Origin><Source>GeometricFeature</Source><FeatureName>bottom surface</FeatureName></Origin><PrimaryAxis><DefinedDirection>+Z</DefinedDirection><Source>ReferenceFrame</Source><SourceDirection>+Z</SourceDirection><FeatureName></FeatureName></PrimaryAxis><SecondaryAxis><DefinedDirection>+X</DefinedDirection><Source>ReferenceFrame</Source><SourceDirection>+X</SourceDirection><FeatureName></FeatureName></SecondaryAxis></Value></Frame><Frame><Id>Frame2</Id><Value><Name>T</Name><Origin><Source>GeometricFeature</Source><FeatureName>top surface</FeatureName></Origin><PrimaryAxis><DefinedDirection>+Z</DefinedDirection><Source>ReferenceFrame</Source><SourceDirection>+Z</SourceDirection><FeatureName></FeatureName></PrimaryAxis><SecondaryAxis><DefinedDirection>+X</DefinedDirection><Source>ReferenceFrame</Source><SourceDirection>+X</SourceDirection><FeatureName></FeatureName></SecondaryAxis></Value></Frame></Frames>
  Post R : sm_lib/Body Elements/Cylindrical Solid  CylinderRadius=post_r  CylinderRadiusUnits=m  CylinderLength=post_h  CylinderLengthUnits=m  ExportEntireGeometry=off  InertiaType=CalculateFromGeometry  BasedOnType=Density  Density=1000  DensityUnits=kg/m^3  Mass=1  MassUnits=kg  CenterOfMass=[0 0 0]  CenterOfMassUnits=m  MomentsOfInertia=[1 1 1]  MomentsOfInertiaUnits=kg*m^2  ProductsOfInertia=[0 0 0]  ProductsOfInertiaUnits=kg*m^2  GraphicType=FromGeometry  MarkerShape=Sphere  MarkerSize=10  GraphicVisPropType=SimpleVisualProperties  GraphicDiffuseColor=post_clr  GraphicOpacity=post_opc  GraphicSpecularColor=[0.5 0.5 0.5 1.0]  GraphicAmbientColor=[0.15 0.15 0.15 1.0]  GraphicEmissiveColor=[0.0 0.0 0.0 1.0]  GraphicShininess=75  DoExposeReferenceFrame=off  SerializedFrames=<Frames><Frame><Id>Frame1</Id><Value><Name>B</Name><Origin><Source>GeometricFeature</Source><FeatureName>bottom surface</FeatureName></Origin><PrimaryAxis><DefinedDirection>+Z</DefinedDirection><Source>ReferenceFrame</Source><SourceDirection>+Z</SourceDirection><FeatureName></FeatureName></PrimaryAxis><SecondaryAxis><DefinedDirection>+X</DefinedDirection><Source>ReferenceFrame</Source><SourceDirection>+X</SourceDirection><FeatureName></FeatureName></SecondaryAxis></Value></Frame><Frame><Id>Frame2</Id><Value><Name>T</Name><Origin><Source>GeometricFeature</Source><FeatureName>top surface</FeatureName></Origin><PrimaryAxis><DefinedDirection>+Z</DefinedDirection><Source>ReferenceFrame</Source><SourceDirection>+Z</SourceDirection><FeatureName></FeatureName></PrimaryAxis><SecondaryAxis><DefinedDirection>+X</DefinedDirection><Source>ReferenceFrame</Source><SourceDirection>+X</SourceDirection><FeatureName></FeatureName></SecondaryAxis></Value></Frame></Frames>
  R1 : Subsystem  mask{square_lwh=[0.01 1 1]}
      mask prompts: square_lwh "Size [l w h] (m)"
  R2 : Subsystem  mask{square_lwh=[0.01 1 1]}
      mask prompts: square_lwh "Size [l w h] (m)"
  R3 : Subsystem  mask{square_lwh=[0.01 1 1]}
      mask prompts: square_lwh "Size [l w h] (m)"
  R4 : Subsystem  mask{square_lwh=[0.01 1 1]}
      mask prompts: square_lwh "Size [l w h] (m)"
  R5 : Subsystem  mask{square_lwh=[0.01 1 1]}
      mask prompts: square_lwh "Size [l w h] (m)"
  Transform Orient Line : sm_lib/Frames and Transforms/Rigid Transform  RotationMethod=RotationSequence  FollAlignAxisA=+X  BaseAlignAxisA=+Y  FollAlignAxisB=+Y  BaseAlignAxisB=+Z  RotationStandardAxis=+Z  RotationAngle=0  RotationAngleUnits=deg  RotationArbitraryAxis=[0 0 1]  RotationSequenceAxes=FollowerAxes  RotationSequence=ZYX  RotationSequenceAngles=[offset_yaw offset_pitch offset_roll]  RotationSequenceAnglesUnits=rad  RotationMatrix=[1 0 0; 0 1 0; 0 0 1]  Quaternion=[1 0 0 0]  TranslationMethod=Cartesian  TranslationCartesianOffset=offset_xyz  TranslationCartesianOffsetUnits=m  TranslationStandardAxis=+Z  TranslationStandardOffset=0  TranslationStandardOffsetUnits=m  TranslationROffset=0  TranslationROffsetUnits=m  TranslationThetaOffset=0  TranslationThetaOffsetUnits=deg  TranslationZOffset=0  TranslationZOffsetUnits=m
  Transform Post L : sm_lib/Frames and Transforms/Rigid Transform  RotationMethod=StandardAxis  FollAlignAxisA=+X  BaseAlignAxisA=+Y  FollAlignAxisB=+Y  BaseAlignAxisB=+Z  RotationStandardAxis=+Y  RotationAngle=0.0  RotationAngleUnits=deg  RotationArbitraryAxis=[0 0 1]  RotationSequenceAxes=FollowerAxes  RotationSequence=XYX  RotationSequenceAngles=[0 0 0]  RotationSequenceAnglesUnits=deg  RotationMatrix=[1 0 0; 0 1 0; 0 0 1]  Quaternion=[1 0 0 0]  TranslationMethod=StandardAxis  TranslationCartesianOffset=[0 0 0]  TranslationCartesianOffsetUnits=m  TranslationStandardAxis=+Y  TranslationStandardOffset=line_w/2  TranslationStandardOffsetUnits=m  TranslationROffset=0  TranslationROffsetUnits=m  TranslationThetaOffset=0  TranslationThetaOffsetUnits=deg  TranslationZOffset=0  TranslationZOffsetUnits=m
  Transform Post R : sm_lib/Frames and Transforms/Rigid Transform  RotationMethod=StandardAxis  FollAlignAxisA=+X  BaseAlignAxisA=+Y  FollAlignAxisB=+Y  BaseAlignAxisB=+Z  RotationStandardAxis=+Y  RotationAngle=0.0  RotationAngleUnits=deg  RotationArbitraryAxis=[0 0 1]  RotationSequenceAxes=FollowerAxes  RotationSequence=XYX  RotationSequenceAngles=[0 0 0]  RotationSequenceAnglesUnits=deg  RotationMatrix=[1 0 0; 0 1 0; 0 0 1]  Quaternion=[1 0 0 0]  TranslationMethod=StandardAxis  TranslationCartesianOffset=[0 0 0]  TranslationCartesianOffsetUnits=m  TranslationStandardAxis=+Y  TranslationStandardOffset=line_w/2  TranslationStandardOffsetUnits=m  TranslationROffset=0  TranslationROffsetUnits=m  TranslationThetaOffset=0  TranslationThetaOffsetUnits=deg  TranslationZOffset=0  TranslationZOffsetUnits=m
  W : PMIOPort  Side=Left
  connections:
  Post R/RConn1 -- R1/RConn1
  R2/RConn1 -- R1/LConn1
  L2/RConn1 -- L3/LConn1
  R4/RConn1 -- R3/LConn1
  Transform Post R/LConn1 -- Post R/LConn1
  L3/RConn1 -- L4/LConn1
  Post L/LConn1 -- Transform Post L/RConn1
  W/RConn1 -- Transform Orient Line/LConn1
  R2/LConn1 -- R3/RConn1
  L5/LConn1 -- L4/RConn1
  R5/RConn1 -- R4/LConn1
  L1/RConn1 -- L2/LConn1
  L1/LConn1 -- Post L/RConn1
  Transform Post L/LConn1 -- Transform Orient Line/RConn1 -- Transform Post R/RConn1

== system sm_car_/World/Scene/CRG Hockenheim F/STL Geometry Centerline ==
  Geometry : sm_lib/Body Elements/File Solid  ExtGeomFileName=CRG_Hockenheim_f_centerline.stl  UnitType=Custom  ExtGeomFileUnits=m  StepReaderType=HEX  ExportConvexHullGeometry=off  InertiaType=Custom  BasedOnType=DensityFromFile  Density=1000  DensityUnits=kg/m^3  Mass=1  MassUnits=kg  CenterOfMass=[0 0 0]  CenterOfMassUnits=m  MomentsOfInertia=[1 1 1]  MomentsOfInertiaUnits=kg*m^2  ProductsOfInertia=[0 0 0]  ProductsOfInertiaUnits=kg*m^2  GraphicType=FromGeometry  MarkerShape=Sphere  MarkerSize=10  GraphicVisPropType=SimpleVisualProperties  GraphicDiffuseColor=stl_clr  GraphicOpacity=stl_opc  GraphicSpecularColor=[0.5 0.5 0.5 1.0]  GraphicAmbientColor=[0.15 0.15 0.15 1.0]  GraphicEmissiveColor=[0.0 0.0 0.0 1.0]  GraphicShininess=75  DoExposeReferenceFrame=on  SerializedFrames=<Frames/>
  Transform Geometry : sm_lib/Frames and Transforms/Rigid Transform  RotationMethod=RotationSequence  FollAlignAxisA=+X  BaseAlignAxisA=+Y  FollAlignAxisB=+Y  BaseAlignAxisB=+Z  RotationStandardAxis=+Z  RotationAngle=0  RotationAngleUnits=rad  RotationArbitraryAxis=[0 0 1]  RotationSequenceAxes=FollowerAxes  RotationSequence=ZYX  RotationSequenceAngles=[stl_yaw stl_pitch stl_roll]  RotationSequenceAnglesUnits=rad  RotationMatrix=[1 0 0; 0 1 0; 0 0 1]  Quaternion=[1 0 0 0]  TranslationMethod=Cartesian  TranslationCartesianOffset=[stl_x stl_y stl_z]  TranslationCartesianOffsetUnits=m  TranslationStandardAxis=+Z  TranslationStandardOffset=0  TranslationStandardOffsetUnits=m  TranslationROffset=0  TranslationROffsetUnits=m  TranslationThetaOffset=0  TranslationThetaOffsetUnits=deg  TranslationZOffset=0  TranslationZOffsetUnits=m
  W : PMIOPort  Side=Right
  connections:
  Geometry/RConn1 -- Transform Geometry/RConn1
  Transform Geometry/LConn1 -- W/RConn1
